simulink model "chaine_qpsk_ham_sim"  (R2023b)
settings: Solver=FixedStepDiscrete  StartTime=0.0  StopTime=Nbq*7  FixedStep=1  RelTol=1e-3
undefined symbols (not defined in the file): dly, sigq2
settings Model: Creator=e2507457  LastModifiedBy=e2507457

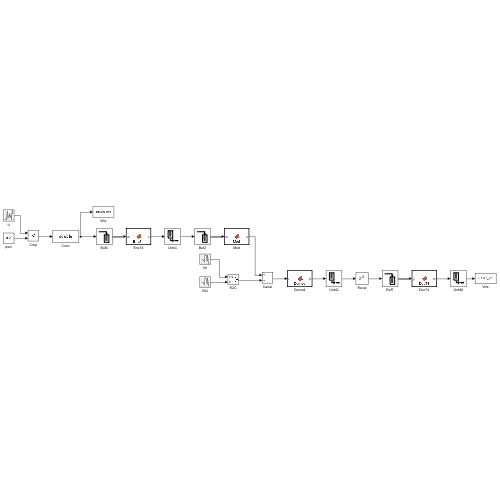
[thumbnail: Simulink's stored preview of the top-level diagram]
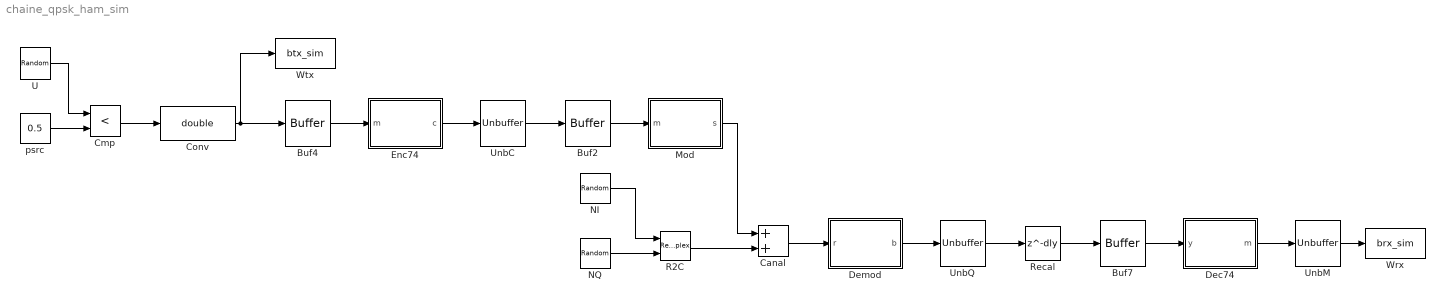
== system chaine_qpsk_ham_sim ==
  Buf2 : Buffer  N=2
  Buf4 : Buffer  N=4
  Buf7 : Buffer  N=7
  Canal : Sum
  Cmp : RelationalOperator  Operator=<  OutDataTypeStr=boolean  RndMeth=Simplest  InputSameDT=off
  Conv : DataTypeConversion  OutDataTypeStr=double  SaturateOnIntegerOverflow=off  RndMeth=Floor
  Dec74 : MATLAB Function  TreatAsAtomicUnit=on
  Demod : MATLAB Function  TreatAsAtomicUnit=on
  Enc74 : MATLAB Function  TreatAsAtomicUnit=on
  Mod : MATLAB Function  TreatAsAtomicUnit=on
  NI : RandomNumber  Variance=sigq2  Seed=29  SampleTime=8
  NQ : RandomNumber  Variance=sigq2  Seed=30  SampleTime=8
  R2C : RealImagToComplex
  Recal : Delay  DelayLength=dly  InitialCondition=0  SampleTime=4
  U : UniformRandomNumber  Minimum=0  Seed=28  SampleTime=7
  UnbC : Unbuffer
  UnbM : Unbuffer
  UnbQ : Unbuffer
  Wrx : ToWorkspace  VariableName=brx_sim  SampleTime=-1
  Wtx : ToWorkspace  VariableName=btx_sim  SampleTime=-1
  psrc : Constant  Value=0.5  SampleTime=7
  wires:
  U/1 -> Cmp/1
  psrc/1 -> Cmp/2
  Mod/1(s) -> Canal/1
  Cmp/1 -> Conv/1
  Conv/1 -> Buf4/1, Wtx/1
  Buf2/1 -> Mod/1(m)
  Buf4/1 -> Enc74/1(m)
  Enc74/1(c) -> UnbC/1
  UnbC/1 -> Buf2/1
  NI/1 -> R2C/1
  NQ/1 -> R2C/2
  R2C/1 -> Canal/2
  Canal/1 -> Demod/1(r)
  Demod/1(b) -> UnbQ/1
  UnbQ/1 -> Recal/1
  Recal/1 -> Buf7/1
  Buf7/1 -> Dec74/1(y)
  Dec74/1(m) -> UnbM/1
  UnbM/1 -> Wrx/1

== matlab function chaine_qpsk_ham_sim/Enc74 ==
  data: m input; c output
function c = Enc74(m)
%#codegen
c = [m(1); m(2); m(3); m(4); ...
     mod(m(1)+m(3)+m(4),2); ...
     mod(m(1)+m(2)+m(3),2); ...
     mod(m(2)+m(3)+m(4),2)];
end

== matlab function chaine_qpsk_ham_sim/Demod ==
  data: r input; b output
function b = Demod(r)
%#codegen
b = [double(real(r) < 0); double(imag(r) < 0)];
end

== matlab function chaine_qpsk_ham_sim/Dec74 ==
  data: y input; m output
function m = Dec74(y)
%#codegen
s0 = mod(y(1)+y(3)+y(4)+y(5), 2);
s1 = mod(y(1)+y(2)+y(3)+y(6), 2);
s2 = mod(y(2)+y(3)+y(4)+y(7), 2);
v  = 4*s0 + 2*s1 + s2;
m  = y(1:4);
if v == 6, m(1) = 1 - m(1); end
if v == 3, m(2) = 1 - m(2); end
if v == 7, m(3) = 1 - m(3); end
if v == 5, m(4) = 1 - m(4); end
end

== matlab function chaine_qpsk_ham_sim/Mod ==
  data: m input; s output
function s = Mod(m)
%#codegen
s = complex((1-2*m(1))/sqrt(2), (1-2*m(2))/sqrt(2));
end
